simulink model "leg"  (R2026a)
settings: Solver=ode4  FixedStep=0.02
values from neighbouring files (symbols this model uses):
  g = 9.81    [legParameters.m]
  ls = 0.4    [legParameters.m]
  m = 4    [legParameters.m]
  mu = 0.45    [legParameters.m]
  omega0 = 0    [legParameters.m]
  phi0 = interp1(timePlot.t, timePlot.phi, t0)    [legParameters.m]
  Thetazz = 0.495    [legParameters.m]
settings Model: Creator=a20887  LastModifiedBy=a20887

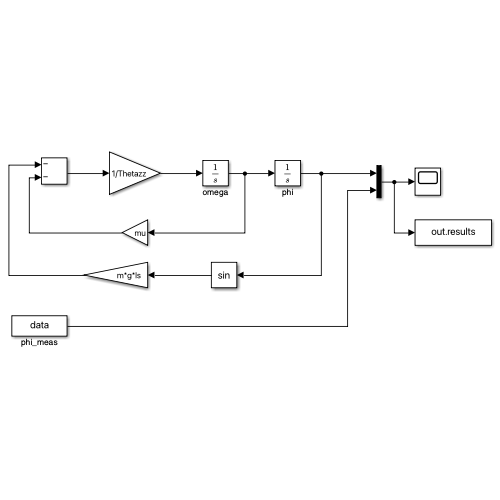
[thumbnail: Simulink's stored preview of the top-level diagram]
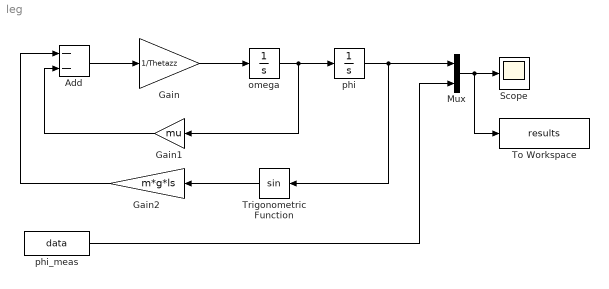
== system leg ==
  Add : Sum  Inputs=--
  Gain : Gain  Gain=1/Thetazz
  Gain1 : Gain  Gain=mu
  Gain2 : Gain  Gain=m*g*ls
  Mux : Mux  Inputs=2
  Scope : Scope
      settings: ActiveDisplayYMinimum=-0.46274952925170865  ActiveDisplayYMaximum=0.58994414717698518
  To Workspace : ToWorkspace  VariableName=results  SaveFormat=Structure With Time  SampleTime=-1
  Trigonometric Function : Trigonometry
  omega : Integrator  InitialCondition=omega0
  phi : Integrator  InitialCondition=phi0
  phi_meas : FromWorkspace  VariableName=data  OutputAfterFinalValue=Holding final value
  wires:
  Add/1 -> Gain/1
  Gain/1 -> omega/1
  omega/1 -> Gain1/1, phi/1
  Trigonometric Function/1 -> Gain2/1
  Gain1/1 -> Add/2
  Gain2/1 -> Add/1
  phi/1 -> Mux/1, Trigonometric Function/1
  phi_meas/1 -> Mux/2
  Mux/1 -> To Workspace/1, Scope/1
